simulink model "Hashimoto"  (R2023a)
settings: Solver=VariableStepAuto  StartTime=0.0  StopTime=2  RelTol=1e-3
libraries: fl_lib x18, nesl_utility x6, slpidlib x1
settings Model: Creator=tessa  LastModifiedBy=carlo

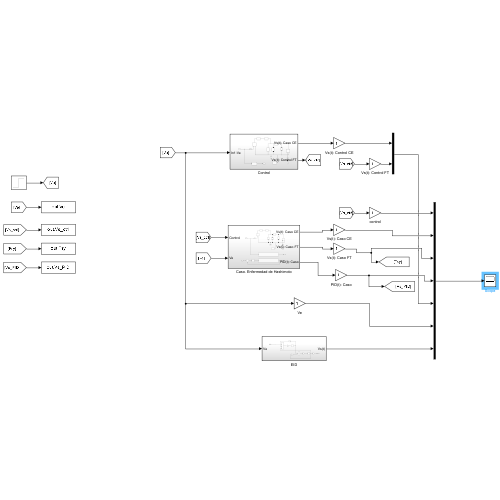
[thumbnail: Simulink's stored preview of the top-level diagram]
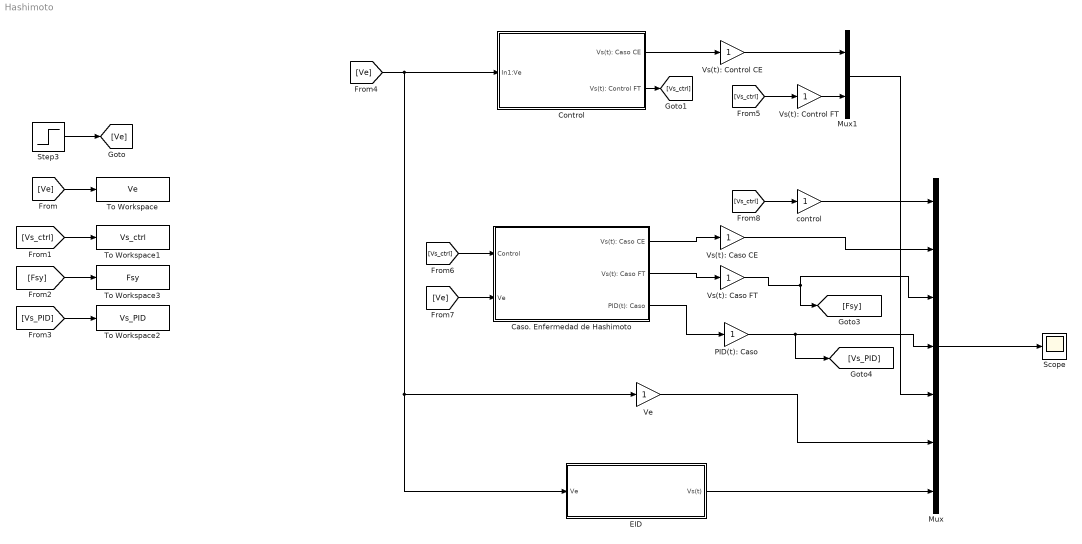
== system Hashimoto ==
  Caso. Enfermedad de Hashimoto : Subsystem
  Control : Subsystem
  EID : Subsystem
  Mux : Mux  Inputs=7
  Mux1 : Mux  Inputs=2
  PID(t): Caso : Gain
  Scope : Scope
  Step3 : Step  Time=0  SampleTime=0
  To Workspace : ToWorkspace  VariableName=Ve  SampleTime=-1
  To Workspace1 : ToWorkspace  VariableName=Vs_ctrl  SampleTime=-1
  To Workspace2 : ToWorkspace  VariableName=Vs_PID  SampleTime=-1
  To Workspace3 : ToWorkspace  VariableName=Fsy  SampleTime=-1
  Ve : Gain
  Vs(t): Caso CE : Gain
  Vs(t): Caso FT : Gain
  Vs(t): Control CE : Gain
  Vs(t): Control FT : Gain
  control : Gain
  wires:
  Step3/1 -> [Ve]
  [Ve] -> To Workspace/1
  [Vs_ctrl] -> To Workspace1/1
  [Fsy] -> To Workspace3/1
  [Vs_PID] -> To Workspace2/1
  [Ve] -> EID/1(Ve), Ve/1, Control/1(In1:Ve)
  Control/1(Vs(t): Caso CE) -> Vs(t): Control CE/1
  Control/2(Vs(t): Control FT) -> [Vs_ctrl]
  Vs(t): Control CE/1 -> Mux1/1
  Vs(t): Control FT/1 -> Mux1/2
  [Vs_ctrl] -> Vs(t): Control FT/1
  [Vs_ctrl] -> Caso. Enfermedad de Hashimoto/1(Control)
  Caso. Enfermedad de Hashimoto/2(Vs(t): Caso FT) -> Vs(t): Caso FT/1
  Caso. Enfermedad de Hashimoto/3(PID(t): Caso) -> PID(t): Caso/1
  PID(t): Caso/1 -> [Vs_PID], Mux/4
  Vs(t): Caso FT/1 -> [Fsy], Mux/3
  Vs(t): Caso CE/1 -> Mux/2
  [Vs_ctrl] -> control/1
  Mux/1 -> Scope/1
  Mux1/1 -> Mux/5
  Caso. Enfermedad de Hashimoto/1(Vs(t): Caso CE) -> Vs(t): Caso CE/1
  [Ve] -> Caso. Enfermedad de Hashimoto/2(Ve)
  Ve/1 -> Mux/6
  control/1 -> Mux/1
  EID/1(Vs(t)) -> Mux/7

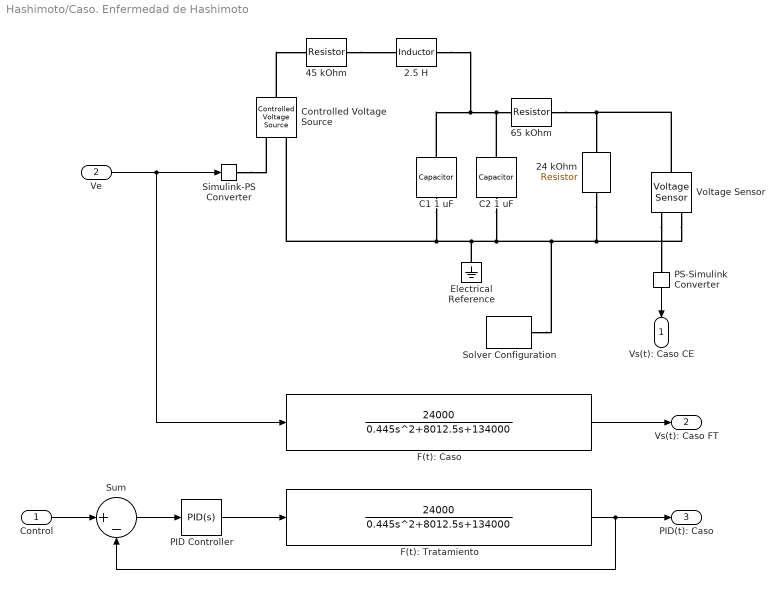
== system Hashimoto/Caso. Enfermedad de Hashimoto ==
  Control : Inport
  Ve : Inport  Port=2
  2.5 H : fl_lib/Electrical/Electrical Elements/Inductor  l=2.5 H  r=0 Ohm  g=1e-9 1/Ohm  i_specify=off  i_priority=None  i=0 A  i_nominal_specify=off  i_nominal_unit=A  i_nominal_value=1  v_specify=off  v_priority=None  v=0 V  v_nominal_specify=off  v_nominal_unit=V  v_nominal_value=1  i_L_specify=off  i_L_priority=High  i_L=0 A  i_L_nominal_specify=off  i_L_nominal_unit=A  i_L_nominal_value=1
  24 kOhm : fl_lib/Electrical/Electrical Elements/Resistor  R=24 kOhm  i_specify=off  i_priority=None  i=0 A  i_nominal_specify=off  i_nominal_unit=A  i_nominal_value=1  v_specify=off  v_priority=None  v=0 V  v_nominal_specify=off  v_nominal_unit=V  v_nominal_value=1
  45 kOhm : fl_lib/Electrical/Electrical Elements/Resistor  R=45 kOhm  i_specify=off  i_priority=None  i=0 A  i_nominal_specify=off  i_nominal_unit=A  i_nominal_value=1  v_specify=off  v_priority=None  v=0 V  v_nominal_specify=off  v_nominal_unit=V  v_nominal_value=1
  65 kOhm : fl_lib/Electrical/Electrical Elements/Resistor  R=65 kOhm  i_specify=off  i_priority=None  i=0 A  i_nominal_specify=off  i_nominal_unit=A  i_nominal_value=1  v_specify=off  v_priority=None  v=0 V  v_nominal_specify=off  v_nominal_unit=V  v_nominal_value=1
  C1 1 uF : fl_lib/Electrical/Electrical Elements/Capacitor  c=1 uF  r=1e-6 Ohm  g=0 1/Ohm  i_specify=off  i_priority=None  i=0 A  i_nominal_specify=off  i_nominal_unit=A  i_nominal_value=1  v_specify=off  v_priority=None  v=0 V  v_nominal_specify=off  v_nominal_unit=V  v_nominal_value=1  vc_specify=off  vc_priority=High  vc=0 V  vc_nominal_specify=off  vc_nominal_unit=V  vc_nominal_value=1
  C2 1 uF : fl_lib/Electrical/Electrical Elements/Capacitor  c=1 uF  r=1e-6 Ohm  g=0 1/Ohm  i_specify=off  i_priority=None  i=0 A  i_nominal_specify=off  i_nominal_unit=A  i_nominal_value=1  v_specify=off  v_priority=None  v=0 V  v_nominal_specify=off  v_nominal_unit=V  v_nominal_value=1  vc_specify=off  vc_priority=High  vc=0 V  vc_nominal_specify=off  vc_nominal_unit=V  vc_nominal_value=1
  Controlled Voltage Source : fl_lib/Electrical/Electrical Sources/Controlled Voltage Source
  Electrical Reference : fl_lib/Electrical/Electrical Elements/Electrical Reference
  F(t): Caso : TransferFcn  Numerator=[24000]  Denominator=[0.445 8012.5 134000]
  F(t): Tratamiento : TransferFcn  Numerator=[24000]  Denominator=[0.445 8012.5 134000]
  PID Controller : slpidlib/PID Controller  Controller=PID  Form=Parallel  TimeDomain=Continuous-time  UseExternalTs=off  SampleTime=-1  IntegratorMethod=Forward Euler  FilterMethod=Forward Euler  ControllerParametersSource=internal  P=2000  I=33480  UseKiTs=off  D=0.1112  N=20000  UseFilter=on  TunerSelectOption=Transfer Function Based (PID Tuner App)  InitialConditionSource=internal  InitialConditionForIntegrator=0  InitialConditionForFilter=0  DifferentiatorICPrevScaledInput=0  ExternalReset=none  TrackingMode=off  Kt=1  LimitOutput=off  SatLimitsSource=internal  UpperSaturationLimit=inf  LowerSaturationLimit=-inf  LinearizeAsGain=on  AntiWindupMode=none  Kb=1  LimitIntegrator=off  UpperIntegratorSaturationLimit=inf  LowerIntegratorSaturationLimit=-inf  POutMin=[]  POutMax=[]  IOutMin=[]  IOutMax=[]  DOutMin=[]  DOutMax=[]  NOutMin=[]  NOutMax=[]  SumOutMin=[]  SumOutMax=[]  SaturationOutMin=[]  SaturationOutMax=[]  PParamMin=[]  PParamMax=[]  IParamMin=[]  IParamMax=[]  DParamMin=[]  DParamMax=[]  NParamMin=[]  NParamMax=[]  KbParamMin=[]  KbParamMax=[]  KtParamMin=[]  KtParamMax=[]  KbOutMin=[]  KbOutMax=[]  KtOutMin=[]  KtOutMax=[]  IntegratorOutMin=[]  IntegratorOutMax=[]  FilterOutMin=[]  FilterOutMax=[]  SumI1OutMin=[]  SumI1OutMax=[]  SumI2OutMin=[]  SumI2OutMax=[]  SumI3OutMin=[]  SumI3OutMax=[]  SumI4OutMin=[]  SumI4OutMax=[]  SumDOutMin=[]  SumDOutMax=[]  DifferentiatorOutMin=[]  DifferentiatorOutMax=[]  FilterDiffOutCoefMin=[]  FilterDiffOutCoefMax=[]  ReciprocalOutMin=[]  ReciprocalOutMax=[]  SumDenOutMin=[]  SumDenOutMax=[]  SumNumOutMin=[]  SumNumOutMax=[]  DivideOutMin=[]  DivideOutMax=[]  UdiffTsProdOutMin=[]  UdiffTsProdOutMax=[]  NTsProdOutMin=[]  NTsProdOutMax=[]  UintegralTsProdOutMin=[]  UintegralTsProdOutMax=[]  UngainTsProdOutMin=[]  UngainTsProdOutMax=[]  ClampingZeroOutDataTypeStr=Inherit: Inherit via back propagation  ClampingZeroOutMin=[]  ClampingZeroOutMax=[]  FilterDenConstantOutDataTypeStr=Inherit: Inherit via back propagation  FilterDenConstantOutMin=[]  FilterDenConstantOutMax=[]  PCopyOutDataTypeStr=Inherit: Inherit via back propagation  PCopyOutMin=[]  PCopyOutMax=[]  NCopyOutDataTypeStr=Inherit: Inherit via back propagation  NCopyOutMin=[]  NCopyOutMax=[]  IntegratorContinuousStateAttributes=''  IntegratorStateMustResolveToSignalObject=off  IntegratorRTWStateStorageClass=Auto  FilterContinuousStateAttributes=''  FilterStateMustResolveToSignalObject=off  FilterRTWStateStorageClass=Auto  ParallelPVariant=InternalParameters  IdealPVariant=Disabled  IVariant=InternalParameters  DVariant=InternalParameters  IntegratorVariant=Continuous  SatVariant=Disabled  AWVariant=Passthrough  PCopyVariant=Disabled  TRVariant=Disabled  FdbkBlocksVariant=Forward  IdealPFdbkVariant=Disabled  SatFdbkVariant=Disabled  DerivativeFilterVariant=ContFilter  NVariant=InternalParameters  NCopyVariant=Disabled  FilterICVariant=InternalICsFilter  IntegratorICVariant=InternalICs  ExternalResetVariant=Disabled  TRSumVariant=Passthrough  SumFdbkVariant=Disabled  SumVariant=Sum_PID  TsampFilterVariant=InternalTs  TsampNgainVariant=Passthrough  TsampIntegralVariant=Disabled_SignalSpec  ExternalSaturationOutDataTypeStr=Inherit: Same as second input
  PS-Simulink Converter : nesl_utility/PS-Simulink Converter  PhysicalDomain=network_engine_domain  SubClassName=ps_output  LeftPortType=input  RightPortType=output  PseudoPeriodic=off  Frequencies=[]  VectorFormat=inherit  Unit=inherit  AffineConversion=off
  Simulink-PS Converter : nesl_utility/Simulink-PS Converter  PhysicalDomain=network_engine_domain  SubClassName=ps_input  LeftPortType=input  RightPortType=output  PseudoPeriodic=off  Frequencies=[]  NoiseDistribution=none  NoiseParameters=[]  Unit=1  AffineConversion=off  FilteringAndDerivatives=provide  SimscapeFilterOrder=1  InputFilterTimeConstant=0.001  UdotUserProvided=0
  Solver Configuration : nesl_utility/Solver Configuration  PhysicalDomain=network_engine_domain  SubClassName=solver  LeftPortType=input  RightPortType=generic  Tones=[]  Harmonics=[]  SimulateNoise=off  Profile=off  UseLocalSampling=off  EnableSwitchedLinearOptims=on  FrequencyDomain=off  UseCCode=off  RelTol=0.001  AbsTol=0.001  MinStep=1e-09  ToWorkspace=off  RevertToSquareIcSolve=off  NumHomotopyIterations=100  PhasorMode=off  PhasorModeNumHarmonics=1  ConsistencySolver=NEWTON_XTOL_AFTER_FTOL  IndexReductionMethod=DerivativeReplacement  DoDC=off  ResidualTolerance=1e-09  ConsistencyTolSource=GLOBAL  ConsistencyAbsTol=0.001  ConsistencyRelTol=0.001  ConsistencyTolFactor=0.001  UseLocalSolver=off  LocalSolverChoice=NE_BACKWARD_EULER_ADVANCER  ResolveIndetEquations=on  FunctionEvalNumThread=1  LocalSolverSampleTime=0.001  DoFixedCost=off  MaxNonlinIter=3  MaxModeIter=2  ComputeImpulses=off  ImpulseIterations=2  LinearAlgebra=auto  LinearAlgebraNumThread=0  EquationFormulation=NE_TIME_EF  DelaysMemoryBudget=1024  AutomaticFiltering=on  FilteringTimeConstant=0.001  PartitionStorageMethod=AS_NEEDED  PartitionMemoryBudget=1024  PartitionMethod=ROBUST
  Sum : Sum  Inputs=|+-
  Voltage Sensor : fl_lib/Electrical/Electrical Sensors/Voltage Sensor
  Vs(t): Caso CE : Outport
  Vs(t): Caso FT : Outport  Port=2
  PID(t): Caso : Outport  Port=3
  wires:
  F(t): Caso/1 -> Vs(t): Caso FT/1
  PID Controller/1 -> F(t): Tratamiento/1
  Control/1 -> Sum/1
  Sum/1 -> PID Controller/1
  F(t): Tratamiento/1 -> PID(t): Caso/1, Sum/2
  Ve/1 -> F(t): Caso/1, Simulink-PS Converter/1
  PS-Simulink Converter/1 -> Vs(t): Caso CE/1
  connections:
  C1 1 uF/LConn1 -- 2.5 H/RConn1 -- C2 1 uF/LConn1 -- 65 kOhm/LConn1
  Voltage Sensor/RConn2 -- 24 kOhm/RConn1 -- Solver Configuration/RConn1 -- C2 1 uF/RConn1 -- Electrical Reference/LConn1 -- C1 1 uF/RConn1 -- Controlled Voltage Source/RConn2
  65 kOhm/RConn1 -- Voltage Sensor/LConn1 -- 24 kOhm/LConn1
  45 kOhm/RConn1 -- 2.5 H/LConn1
  Simulink-PS Converter/RConn1 -- Controlled Voltage Source/RConn1
  Controlled Voltage Source/LConn1 -- 45 kOhm/LConn1
  Voltage Sensor/RConn1 -- PS-Simulink Converter/LConn1

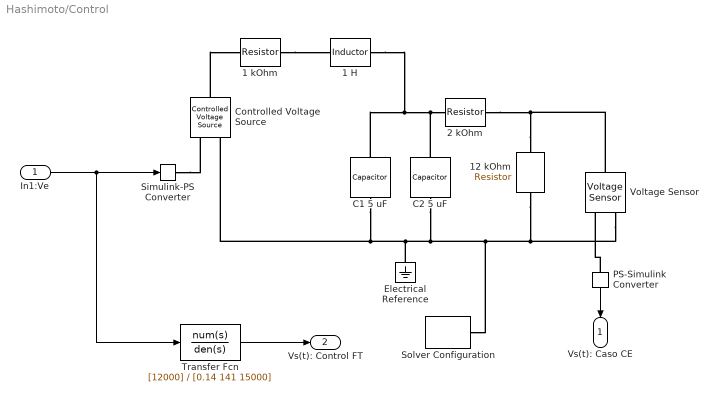
== system Hashimoto/Control ==
  In1:Ve : Inport
  1 H : fl_lib/Electrical/Electrical Elements/Inductor  l=1 H  r=0 Ohm  g=1e-9 1/Ohm  i_specify=off  i_priority=None  i=0 A  i_nominal_specify=off  i_nominal_unit=A  i_nominal_value=1  v_specify=off  v_priority=None  v=0 V  v_nominal_specify=off  v_nominal_unit=V  v_nominal_value=1  i_L_specify=off  i_L_priority=High  i_L=0 A  i_L_nominal_specify=off  i_L_nominal_unit=A  i_L_nominal_value=1
  1 kOhm : fl_lib/Electrical/Electrical Elements/Resistor  R=1 kOhm  i_specify=off  i_priority=None  i=0 A  i_nominal_specify=off  i_nominal_unit=A  i_nominal_value=1  v_specify=off  v_priority=None  v=0 V  v_nominal_specify=off  v_nominal_unit=V  v_nominal_value=1
  12 kOhm : fl_lib/Electrical/Electrical Elements/Resistor  R=12 kOhm  i_specify=off  i_priority=None  i=0 A  i_nominal_specify=off  i_nominal_unit=A  i_nominal_value=1  v_specify=off  v_priority=None  v=0 V  v_nominal_specify=off  v_nominal_unit=V  v_nominal_value=1
  2 kOhm : fl_lib/Electrical/Electrical Elements/Resistor  R=2 kOhm  i_specify=off  i_priority=None  i=0 A  i_nominal_specify=off  i_nominal_unit=A  i_nominal_value=1  v_specify=off  v_priority=None  v=0 V  v_nominal_specify=off  v_nominal_unit=V  v_nominal_value=1
  C1 5 uF : fl_lib/Electrical/Electrical Elements/Capacitor  c=5 uF  r=1e-6 Ohm  g=0 1/Ohm  i_specify=off  i_priority=None  i=0 A  i_nominal_specify=off  i_nominal_unit=A  i_nominal_value=1  v_specify=off  v_priority=None  v=0 V  v_nominal_specify=off  v_nominal_unit=V  v_nominal_value=1  vc_specify=off  vc_priority=High  vc=0 V  vc_nominal_specify=off  vc_nominal_unit=V  vc_nominal_value=1
  C2 5 uF : fl_lib/Electrical/Electrical Elements/Capacitor  c=5 uF  r=1e-6 Ohm  g=0 1/Ohm  i_specify=off  i_priority=None  i=0 A  i_nominal_specify=off  i_nominal_unit=A  i_nominal_value=1  v_specify=off  v_priority=None  v=0 V  v_nominal_specify=off  v_nominal_unit=V  v_nominal_value=1  vc_specify=off  vc_priority=High  vc=0 V  vc_nominal_specify=off  vc_nominal_unit=V  vc_nominal_value=1
  Controlled Voltage Source : fl_lib/Electrical/Electrical Sources/Controlled Voltage Source
  Electrical Reference : fl_lib/Electrical/Electrical Elements/Electrical Reference
  PS-Simulink Converter : nesl_utility/PS-Simulink Converter  PhysicalDomain=network_engine_domain  SubClassName=ps_output  LeftPortType=input  RightPortType=output  PseudoPeriodic=off  Frequencies=[]  VectorFormat=inherit  Unit=inherit  AffineConversion=off
  Simulink-PS Converter : nesl_utility/Simulink-PS Converter  PhysicalDomain=network_engine_domain  SubClassName=ps_input  LeftPortType=input  RightPortType=output  PseudoPeriodic=off  Frequencies=[]  NoiseDistribution=none  NoiseParameters=[]  Unit=1  AffineConversion=off  FilteringAndDerivatives=provide  SimscapeFilterOrder=1  InputFilterTimeConstant=0.001  UdotUserProvided=0
  Solver Configuration : nesl_utility/Solver Configuration  PhysicalDomain=network_engine_domain  SubClassName=solver  LeftPortType=input  RightPortType=generic  Tones=[]  Harmonics=[]  SimulateNoise=off  Profile=off  UseLocalSampling=off  EnableSwitchedLinearOptims=on  FrequencyDomain=off  UseCCode=off  RelTol=0.001  AbsTol=0.001  MinStep=1e-09  ToWorkspace=off  RevertToSquareIcSolve=off  NumHomotopyIterations=100  PhasorMode=off  PhasorModeNumHarmonics=1  ConsistencySolver=NEWTON_XTOL_AFTER_FTOL  IndexReductionMethod=DerivativeReplacement  DoDC=off  ResidualTolerance=1e-09  ConsistencyTolSource=GLOBAL  ConsistencyAbsTol=0.001  ConsistencyRelTol=0.001  ConsistencyTolFactor=0.001  UseLocalSolver=off  LocalSolverChoice=NE_BACKWARD_EULER_ADVANCER  ResolveIndetEquations=on  FunctionEvalNumThread=1  LocalSolverSampleTime=0.001  DoFixedCost=off  MaxNonlinIter=3  MaxModeIter=2  ComputeImpulses=off  ImpulseIterations=2  LinearAlgebra=auto  LinearAlgebraNumThread=0  EquationFormulation=NE_TIME_EF  DelaysMemoryBudget=1024  AutomaticFiltering=on  FilteringTimeConstant=0.001  PartitionStorageMethod=AS_NEEDED  PartitionMemoryBudget=1024  PartitionMethod=ROBUST
  Transfer Fcn : TransferFcn  Numerator=[12000]  Denominator=[0.14 141 15000]
  Voltage Sensor : fl_lib/Electrical/Electrical Sensors/Voltage Sensor
  Vs(t): Caso CE : Outport
  Vs(t): Control FT : Outport  Port=2
  wires:
  In1:Ve/1 -> Transfer Fcn/1, Simulink-PS Converter/1
  Transfer Fcn/1 -> Vs(t): Control FT/1
  PS-Simulink Converter/1 -> Vs(t): Caso CE/1
  connections:
  Controlled Voltage Source/RConn2 -- C1 5 uF/RConn1 -- Electrical Reference/LConn1 -- C2 5 uF/RConn1 -- Solver Configuration/RConn1 -- Voltage Sensor/RConn2 -- 12 kOhm/RConn1
  12 kOhm/LConn1 -- 2 kOhm/RConn1 -- Voltage Sensor/LConn1
  2 kOhm/LConn1 -- C1 5 uF/LConn1 -- 1 H/RConn1 -- C2 5 uF/LConn1
  Simulink-PS Converter/RConn1 -- Controlled Voltage Source/RConn1
  Controlled Voltage Source/LConn1 -- 1 kOhm/LConn1
  1 kOhm/RConn1 -- 1 H/LConn1
  PS-Simulink Converter/LConn1 -- Voltage Sensor/RConn1

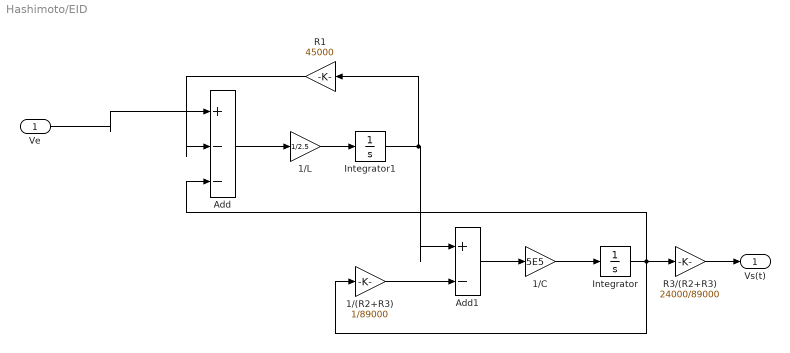
== system Hashimoto/EID ==
  Ve : Inport
  1/(R2+R3) : Gain  Gain=1/89000
  1/C : Gain  Gain=5E5
  1/L : Gain  Gain=1/2.5
  Add : Sum  Inputs=|+--
  Add1 : Sum  Inputs=|+-
  Integrator : Integrator
  Integrator1 : Integrator
  R1 : Gain  Gain=45000
  R3/(R2+R3) : Gain  Gain=24000/89000
  Vs(t) : Outport
  wires:
  R3/(R2+R3)/1 -> Vs(t)/1
  1/(R2+R3)/1 -> Add1/2
  Integrator/1 -> Add/3, 1/(R2+R3)/1, R3/(R2+R3)/1
  R1/1 -> Add/2
  Ve/1 -> Add/1
  1/L/1 -> Integrator1/1
  Integrator1/1 -> R1/1, Add1/1
  Add/1 -> 1/L/1
  1/C/1 -> Integrator/1
  Add1/1 -> 1/C/1
